simulink model "FMT_PlantRHS"  (R2026b)
settings: Solver=FixedStepDiscrete  StopTime=2  FixedStep=0.0005
settings Model: DataDictionary=Flight_Parameters.sldd  Creator=26718  LastModifiedBy=26718

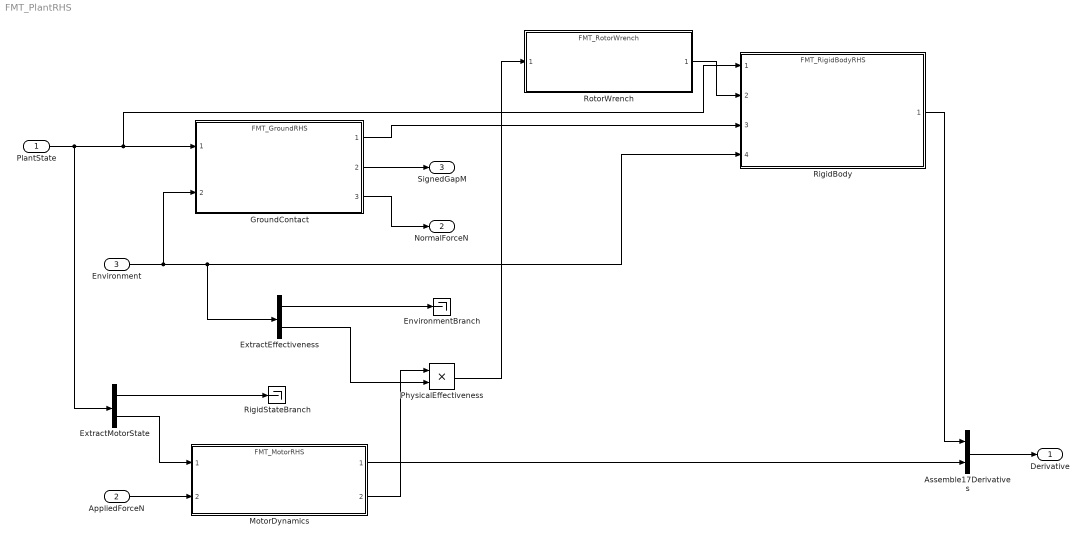
== system FMT_PlantRHS ==
  PlantState : Inport  OutDataTypeStr=double  PortDimensions=17
  AppliedForceN : Inport  Port=2  OutDataTypeStr=double  PortDimensions=4
  Environment : Inport  Port=3  OutDataTypeStr=double  PortDimensions=15
  Assemble17Derivatives : Mux  Inputs=2
  EnvironmentBranch : Terminator
  ExtractEffectiveness : Demux  Outputs=[11 4]
  ExtractMotorState : Demux  Outputs=[13 4]
  GroundContact : ModelReference  ModelNameDialog=FMT_GroundRHS  SimulationMode=Normal  ModelReferenceVersion=1.1
  MotorDynamics : ModelReference  ModelNameDialog=FMT_MotorRHS  SimulationMode=Normal  ModelReferenceVersion=1.1
  PhysicalEffectiveness : Product  Inputs=**
  RigidBody : ModelReference  ModelNameDialog=FMT_RigidBodyRHS  SimulationMode=Normal  ModelReferenceVersion=1.1
  RigidStateBranch : Terminator
  RotorWrench : ModelReference  ModelNameDialog=FMT_RotorWrench  SimulationMode=Normal  ModelReferenceVersion=1.1
  Derivative : Outport
  NormalForceN : Outport  Port=2
  SignedGapM : Outport  Port=3
  wires:
  GroundContact/2 -> SignedGapM/1
  GroundContact/3 -> NormalForceN/1
  Assemble17Derivatives/1 -> Derivative/1
  MotorDynamics/1 -> Assemble17Derivatives/2
  RigidBody/1 -> Assemble17Derivatives/1
  GroundContact/1 -> RigidBody/3
  RotorWrench/1 -> RigidBody/2
  PhysicalEffectiveness/1 -> RotorWrench/1
  MotorDynamics/2 -> PhysicalEffectiveness/1
  AppliedForceN/1 -> MotorDynamics/2
  ExtractEffectiveness/2 -> PhysicalEffectiveness/2
  ExtractEffectiveness/1 -> EnvironmentBranch/1
  Environment/1 -> ExtractEffectiveness/1, RigidBody/4, GroundContact/2
  ExtractMotorState/2 -> MotorDynamics/1
  ExtractMotorState/1 -> RigidStateBranch/1
  PlantState/1 -> GroundContact/1, RigidBody/1, ExtractMotorState/1
